simulink model "hamming_dec_sl"  (R2026b)
settings: Solver=FixedStepDiscrete  FixedStep=1
settings Model: Creator=INS NAWEL  LastModifiedBy=INS NAWEL

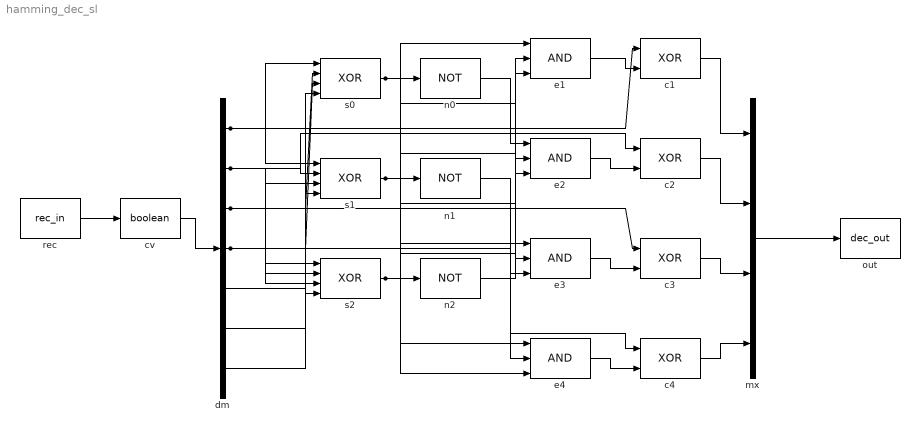
== system hamming_dec_sl ==
  c{1..4} (4 alike) : Logic  Operator=XOR  AllPortsSameDT=off  OutDataTypeStr=boolean
  cv : DataTypeConversion  OutDataTypeStr=boolean  SaturateOnIntegerOverflow=off  RndMeth=Floor
  dm : Demux  Outputs=7
  e{1..4} (4 alike) : Logic  Inputs=3  AllPortsSameDT=off  OutDataTypeStr=boolean
  mx : Mux
  n0 : Logic  Operator=NOT  Inputs=1  AllPortsSameDT=off  OutDataTypeStr=boolean
  n1 : Logic  Operator=NOT  Inputs=1  AllPortsSameDT=off  OutDataTypeStr=boolean
  n2 : Logic  Operator=NOT  Inputs=1  AllPortsSameDT=off  OutDataTypeStr=boolean
  out : ToWorkspace  VariableName=dec_out  SampleTime=1
  rec : FromWorkspace  VariableName=rec_in  SampleTime=1
  s0 : Logic  Operator=XOR  Inputs=4  AllPortsSameDT=off  OutDataTypeStr=boolean
  s1 : Logic  Operator=XOR  Inputs=4  AllPortsSameDT=off  OutDataTypeStr=boolean
  s2 : Logic  Operator=XOR  Inputs=4  AllPortsSameDT=off  OutDataTypeStr=boolean
  wires:
  rec/1 -> cv/1
  cv/1 -> dm/1
  dm/1 -> s0/1, s1/1, c1/1
  dm/3 -> s0/2, s1/3, s2/2, c3/1
  dm/4 -> s0/3, s2/3, c4/1
  dm/5 -> s0/4
  dm/2 -> s1/2, s2/1, c2/1
  dm/6 -> s1/4
  dm/7 -> s2/4
  s0/1 -> n0/1, e1/1, e3/1, e4/1
  s1/1 -> n1/1, e1/2, e2/2, e3/2
  s2/1 -> n2/1, e2/3, e3/3, e4/3
  n2/1 -> e1/3
  n0/1 -> e2/1
  n1/1 -> e4/2
  e1/1 -> c1/2
  e2/1 -> c2/2
  e3/1 -> c3/2
  e4/1 -> c4/2
  c1/1 -> mx/1
  c2/1 -> mx/2
  c3/1 -> mx/3
  c4/1 -> mx/4
  mx/1 -> out/1
